simulink model "usv_3dof_openloop"  (R2024b)
settings: Solver=ode4  StartTime=0  StopTime=12  FixedStep=0.01  RelTol=1e-3
settings Model: Creator=qianr  LastModifiedBy=qianr
settings DataIOCC: SaveOutput=off  SignalLogging=off

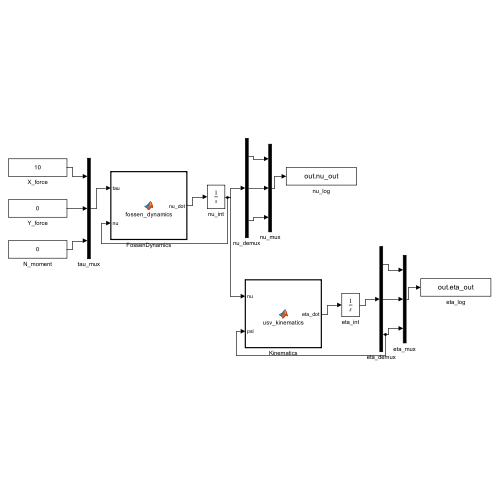
[thumbnail: Simulink's stored preview of the top-level diagram]
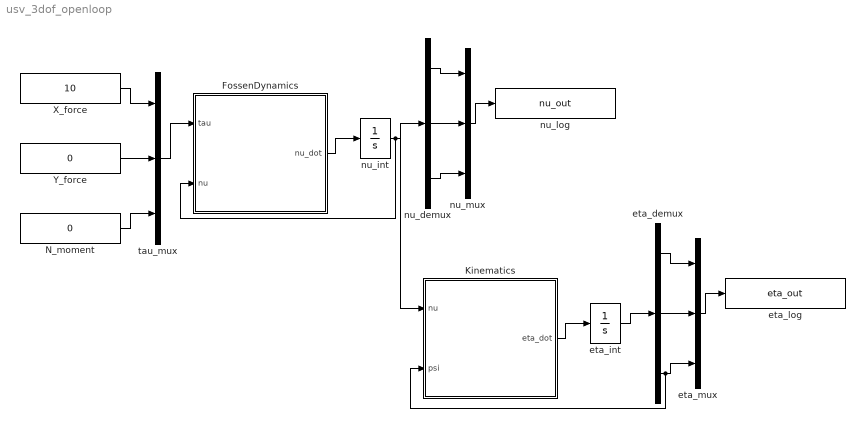
== system usv_3dof_openloop ==
  FossenDynamics : MATLAB Function  TreatAsAtomicUnit=on
  Kinematics : MATLAB Function  TreatAsAtomicUnit=on
  N_moment : Constant  Value=0
  X_force : Constant  Value=10
  Y_force : Constant  Value=0
  eta_demux : Demux  Outputs=3
  eta_int : Integrator  InitialCondition=[0;0;0]
  eta_log : ToWorkspace  VariableName=eta_out  SaveFormat=Timeseries  SampleTime=-1
  eta_mux : Mux  Inputs=3
  nu_demux : Demux  Outputs=3
  nu_int : Integrator  InitialCondition=[0;0;0]
  nu_log : ToWorkspace  VariableName=nu_out  SaveFormat=Timeseries  SampleTime=-1
  nu_mux : Mux  Inputs=3
  tau_mux : Mux  Inputs=3
  wires:
  X_force/1 -> tau_mux/1
  Y_force/1 -> tau_mux/2
  N_moment/1 -> tau_mux/3
  tau_mux/1 -> FossenDynamics/1(tau)
  FossenDynamics/1(nu_dot) -> nu_int/1
  nu_int/1 -> nu_demux/1, FossenDynamics/2(nu), Kinematics/1(nu)
  Kinematics/1(eta_dot) -> eta_int/1
  eta_int/1 -> eta_demux/1
  eta_demux/3 -> Kinematics/2(psi), eta_mux/3
  nu_demux/1 -> nu_mux/1
  nu_demux/2 -> nu_mux/2
  nu_demux/3 -> nu_mux/3
  nu_mux/1 -> nu_log/1
  eta_demux/1 -> eta_mux/1
  eta_demux/2 -> eta_mux/2
  eta_mux/1 -> eta_log/1

== matlab function usv_3dof_openloop/FossenDynamics ==
  data: tau input; nu_dot output; nu input
function nu_dot = fossen_dynamics(tau, nu)
%#codegen
% 三自由度 Fossen 动力学：M*nu_dot = tau - C(nu)*nu - D*nu
m11 = 40; m22 = 50; m33 = 12;
d11 = 8; d22 = 25; d33 = 25;
X = tau(1); Y = tau(2); N = tau(3);
u = nu(1); v = nu(2); r = nu(3);
u_dot = (X + m22*v*r - d11*u) / m11;
v_dot = (Y - m11*u*r - d22*v) / m22;
r_dot = (N - d33*r) / m33;
nu_dot = [u_dot; v_dot; r_dot];

== matlab function usv_3dof_openloop/Kinematics ==
  data: nu input; eta_dot output; psi input
function eta_dot = usv_kinematics(nu, psi)
%#codegen
% 三自由度运动学：eta_dot = R(psi)*nu
u = nu(1); v = nu(2); r = nu(3);
eta_dot = [ u*cos(psi) - v*sin(psi);
            u*sin(psi) + v*cos(psi);
            r ];
